simulink model "chaine_P5c"  (R2023b)
settings: Solver=FixedStepDiscrete  StartTime=0.0  StopTime=10.0  RelTol=1e-3
values from neighbouring files (symbols this model uses):
  D6 = NaN    [partie5_q6.m]
  K7c = mod(-dc, 7)    [partie5_q6.m]
undefined symbols (not defined in the file or in its folder): graine, graine_bruit, nErrMax, sigma2, tab_b1, tab_b2, tab_I, tab_Q, Tb, Tc, Ts_c
libraries: simulink x8
settings Model: Creator=e2405714  LastModifiedBy=e2405714

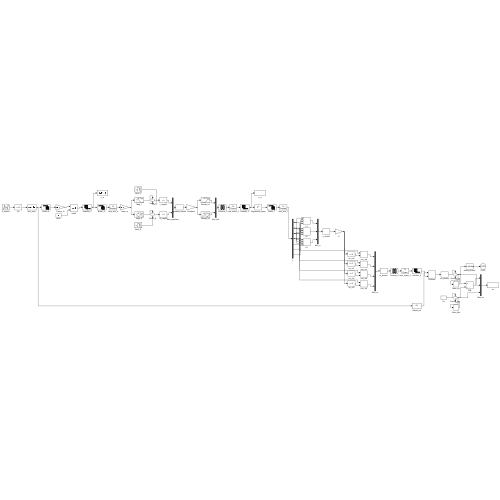
[thumbnail: Simulink's stored preview of the top-level diagram]
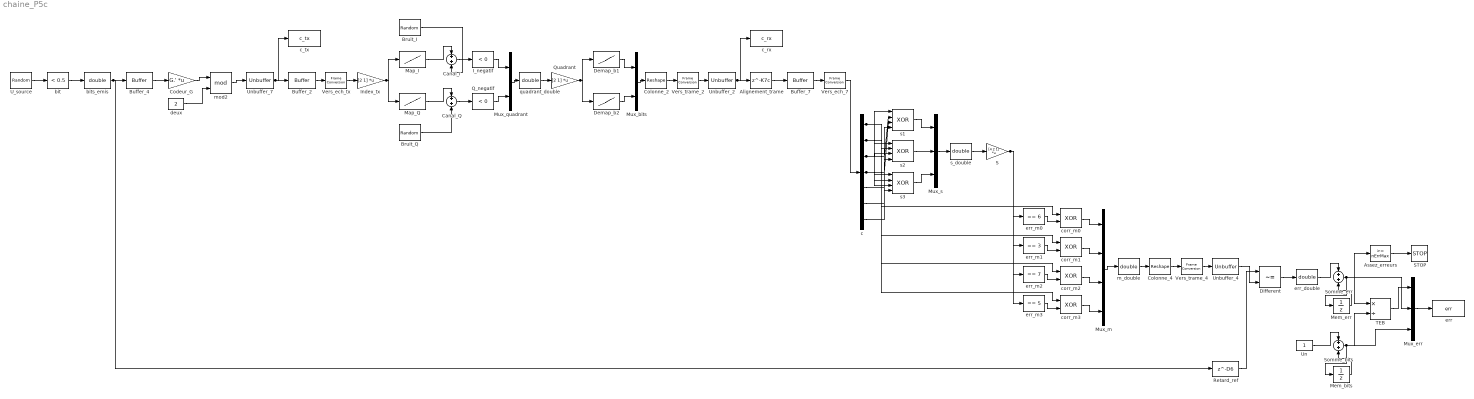
== system chaine_P5c ==
  Alignement_trame : Delay  DelayLength=K7c  SampleTime=Tc
  Assez_erreurs : simulink/Logic and Bit Operations/Compare To Constant  relop=>=  const=nErrMax  OutDataTypeStr=boolean
  Bruit_I : RandomNumber  Variance=sigma2  Seed=graine_bruit  SampleTime=Ts_c
  Bruit_Q : RandomNumber  Variance=sigma2  Seed=graine_bruit + 1  SampleTime=Ts_c
  Buffer_2 : Buffer  N=2
  Buffer_4 : Buffer  N=4
  Buffer_7 : Buffer  N=7
  Canal_I : Sum
  Canal_Q : Sum
  Codeur_G : Gain  Gain=G.'  Multiplication=Matrix(K*u)
  Colonne_2 : Reshape  OutputDimensionality=Column vector (2-D)
  Colonne_4 : Reshape  OutputDimensionality=Column vector (2-D)
  Demap_b1 : Lookup_n-D  NumberOfTableDimensions=1  BreakpointsForDimension1=0:3  Table=tab_b1  InternalRulePriority=Speed  RndMeth=Simplest
  Demap_b2 : Lookup_n-D  NumberOfTableDimensions=1  BreakpointsForDimension1=0:3  Table=tab_b2  InternalRulePriority=Speed  RndMeth=Simplest
  Different : RelationalOperator  Operator=~=  OutDataTypeStr=boolean  RndMeth=Simplest  InputSameDT=off
  I_negatif : simulink/Logic and Bit Operations/Compare To Constant  relop=<  const=0  OutDataTypeStr=boolean
  Index_tx : Gain  Gain=[2 1]  Multiplication=Matrix(K*u)
  Map_I : Lookup_n-D  NumberOfTableDimensions=1  BreakpointsForDimension1=0:3  Table=tab_I  InternalRulePriority=Speed  RndMeth=Simplest
  Map_Q : Lookup_n-D  NumberOfTableDimensions=1  BreakpointsForDimension1=0:3  Table=tab_Q  InternalRulePriority=Speed  RndMeth=Simplest
  Mem_bits : UnitDelay  SampleTime=Tb  HasFrameUpgradeWarning=on
  Mem_err : UnitDelay  SampleTime=Tb  HasFrameUpgradeWarning=on
  Mux_bits : Mux  Inputs=2
  Mux_err : Mux  Inputs=3
  Mux_m : Mux
  Mux_quadrant : Mux  Inputs=2
  Mux_s : Mux  Inputs=3
  Q_negatif : simulink/Logic and Bit Operations/Compare To Constant  relop=<  const=0  OutDataTypeStr=boolean
  Quadrant : Gain  Gain=[2 1]  Multiplication=Matrix(K*u)
  Retard_ref : Delay  DelayLength=D6  SampleTime=Tb
  S : Gain  Gain=[4 2 1]  Multiplication=Matrix(K*u)
  STOP : Stop
  Somme_bits : Sum
  Somme_err : Sum
  TEB : Product  Inputs=*/
  U_source : UniformRandomNumber  Minimum=0  Seed=graine  SampleTime=Tb
  Un : Constant  SampleTime=Tb
  Unbuffer_2 : Unbuffer
  Unbuffer_4 : Unbuffer
  Unbuffer_7 : Unbuffer
  Vers_ech_7 : FrameConversion  OutFrame=Sample-based
  Vers_ech_tx : FrameConversion  OutFrame=Sample-based
  Vers_trame_2 : FrameConversion
  Vers_trame_4 : FrameConversion
  bit : simulink/Logic and Bit Operations/Compare To Constant  relop=<  const=0.5  OutDataTypeStr=boolean
  bits_emis : DataTypeConversion  OutDataTypeStr=double  SaturateOnIntegerOverflow=off  RndMeth=Floor
  c : Demux  Outputs=7
  c_rx : ToWorkspace  VariableName=c_rx  SampleTime=-1
  c_tx : ToWorkspace  VariableName=c_tx  SampleTime=-1
  corr_m{0..3} (4 alike) : Logic  Operator=XOR  AllPortsSameDT=off  OutDataTypeStr=boolean
  deux : Constant  Value=2
  err : ToWorkspace  VariableName=err  SampleTime=-1
  err_double : DataTypeConversion  OutDataTypeStr=double  SaturateOnIntegerOverflow=off  RndMeth=Floor
  err_m0 : simulink/Logic and Bit Operations/Compare To Constant  relop===  const=6  OutDataTypeStr=boolean
  err_m1 : simulink/Logic and Bit Operations/Compare To Constant  relop===  const=3  OutDataTypeStr=boolean
  err_m2 : simulink/Logic and Bit Operations/Compare To Constant  relop===  const=7  OutDataTypeStr=boolean
  err_m3 : simulink/Logic and Bit Operations/Compare To Constant  relop===  const=5  OutDataTypeStr=boolean
  m_double : DataTypeConversion  OutDataTypeStr=double  SaturateOnIntegerOverflow=off  RndMeth=Floor
  mod2 : Math  Operator=mod
  quadrant_double : DataTypeConversion  OutDataTypeStr=double  SaturateOnIntegerOverflow=off  RndMeth=Floor
  s1 : Logic  Operator=XOR  Inputs=4  AllPortsSameDT=off  OutDataTypeStr=boolean
  s2 : Logic  Operator=XOR  Inputs=4  AllPortsSameDT=off  OutDataTypeStr=boolean
  s3 : Logic  Operator=XOR  Inputs=4  AllPortsSameDT=off  OutDataTypeStr=boolean
  s_double : DataTypeConversion  OutDataTypeStr=double  SaturateOnIntegerOverflow=off  RndMeth=Floor
  wires:
  U_source/1 -> bit/1
  bit/1 -> bits_emis/1
  bits_emis/1 -> Buffer_4/1, Retard_ref/1
  Buffer_4/1 -> Codeur_G/1
  Codeur_G/1 -> mod2/1
  deux/1 -> mod2/2
  mod2/1 -> Unbuffer_7/1
  Unbuffer_7/1 -> c_tx/1, Buffer_2/1
  Buffer_2/1 -> Vers_ech_tx/1
  Vers_ech_tx/1 -> Index_tx/1
  Index_tx/1 -> Map_I/1, Map_Q/1
  Map_I/1 -> Canal_I/1
  Bruit_I/1 -> Canal_I/2
  Map_Q/1 -> Canal_Q/1
  Bruit_Q/1 -> Canal_Q/2
  Canal_I/1 -> I_negatif/1
  Canal_Q/1 -> Q_negatif/1
  I_negatif/1 -> Mux_quadrant/1
  Q_negatif/1 -> Mux_quadrant/2
  Mux_quadrant/1 -> quadrant_double/1
  quadrant_double/1 -> Quadrant/1
  Quadrant/1 -> Demap_b1/1, Demap_b2/1
  Demap_b1/1 -> Mux_bits/1
  Demap_b2/1 -> Mux_bits/2
  Mux_bits/1 -> Colonne_2/1
  Colonne_2/1 -> Vers_trame_2/1
  Vers_trame_2/1 -> Unbuffer_2/1
  Unbuffer_2/1 -> c_rx/1, Alignement_trame/1
  Alignement_trame/1 -> Buffer_7/1
  Buffer_7/1 -> Vers_ech_7/1
  Vers_ech_7/1 -> c/1
  c/1 -> s1/1, s2/1, corr_m0/1
  c/3 -> s1/2, s2/3, s3/2, corr_m2/1
  c/4 -> s1/3, s3/3, corr_m3/1
  c/5 -> s1/4
  c/2 -> s2/2, s3/1, corr_m1/1
  c/6 -> s2/4
  c/7 -> s3/4
  s1/1 -> Mux_s/1
  s2/1 -> Mux_s/2
  s3/1 -> Mux_s/3
  Mux_s/1 -> s_double/1
  s_double/1 -> S/1
  S/1 -> err_m0/1, err_m1/1, err_m2/1, err_m3/1
  err_m0/1 -> corr_m0/2
  corr_m0/1 -> Mux_m/1
  err_m1/1 -> corr_m1/2
  corr_m1/1 -> Mux_m/2
  err_m2/1 -> corr_m2/2
  corr_m2/1 -> Mux_m/3
  err_m3/1 -> corr_m3/2
  corr_m3/1 -> Mux_m/4
  Mux_m/1 -> m_double/1
  m_double/1 -> Colonne_4/1
  Colonne_4/1 -> Vers_trame_4/1
  Vers_trame_4/1 -> Unbuffer_4/1
  Retard_ref/1 -> Different/1
  Unbuffer_4/1 -> Different/2
  Different/1 -> err_double/1
  err_double/1 -> Somme_err/1
  Mem_err/1 -> Somme_err/2
  Somme_err/1 -> Mem_err/1, TEB/1, Mux_err/2, Assez_erreurs/1
  Un/1 -> Somme_bits/1
  Mem_bits/1 -> Somme_bits/2
  Somme_bits/1 -> Mem_bits/1, TEB/2, Mux_err/3
  TEB/1 -> Mux_err/1
  Mux_err/1 -> err/1
  Assez_erreurs/1 -> STOP/1
